simulink model "Compliance_Front_Axle_"  (R2026a)
settings: Solver=ode23t  StopTime=2
undefined symbols (not defined in the file or in its folder): Camber_Clearance_Coeff, Freeplay_Damping, Freeplay_Stiffness, Freeplay_Threshold, Jounce_Clearance_Coeff, Nominal_Clearance, Steer_Clearance_Coeff, X, Y, Z
libraries: sm_lib x5, nesl_utility x3
settings Model: Creator=Milán  LastModifiedBy=Milán

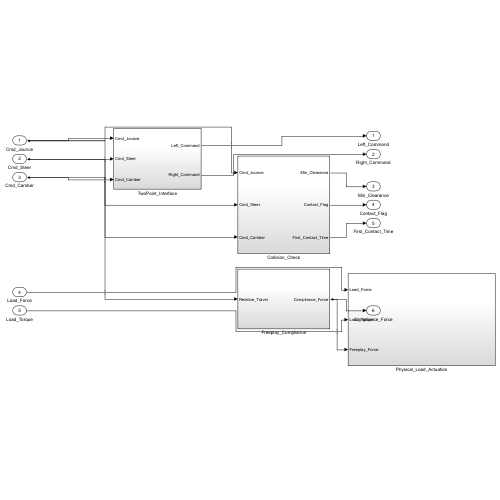
[thumbnail: Simulink's stored preview of the top-level diagram]
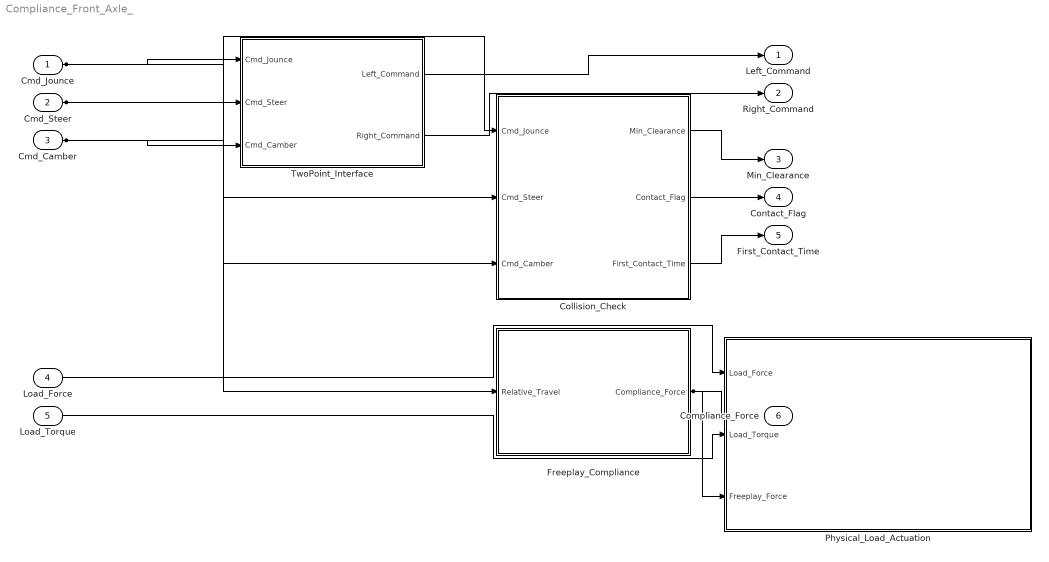
== system Compliance_Front_Axle_ ==
  Cmd_Jounce : Inport
  Cmd_Steer : Inport  Port=2
  Cmd_Camber : Inport  Port=3
  Load_Force : Inport  Port=4  PortDimensions=3
  Load_Torque : Inport  Port=5  PortDimensions=3
  Collision_Check : Subsystem
  Freeplay_Compliance : Subsystem
  Physical_Load_Actuation : Subsystem
  TwoPoint_Interface : Subsystem
  Left_Command : Outport
  Right_Command : Outport  Port=2
  Min_Clearance : Outport  Port=3
  Contact_Flag : Outport  Port=4
  First_Contact_Time : Outport  Port=5
  Compliance_Force : Outport  Port=6
  wires:
  Cmd_Jounce/1 -> TwoPoint_Interface/1(Cmd_Jounce), Collision_Check/1(Cmd_Jounce), Freeplay_Compliance/1(Relative_Travel)
  Cmd_Steer/1 -> TwoPoint_Interface/2(Cmd_Steer), Collision_Check/2(Cmd_Steer)
  Cmd_Camber/1 -> TwoPoint_Interface/3(Cmd_Camber), Collision_Check/3(Cmd_Camber)
  TwoPoint_Interface/1(Left_Command) -> Left_Command/1
  TwoPoint_Interface/2(Right_Command) -> Right_Command/1
  Collision_Check/1(Min_Clearance) -> Min_Clearance/1
  Collision_Check/2(Contact_Flag) -> Contact_Flag/1
  Collision_Check/3(First_Contact_Time) -> First_Contact_Time/1
  Freeplay_Compliance/1(Compliance_Force) -> Compliance_Force/1, Physical_Load_Actuation/3(Freeplay_Force)
  Load_Force/1 -> Physical_Load_Actuation/1(Load_Force)
  Load_Torque/1 -> Physical_Load_Actuation/2(Load_Torque)

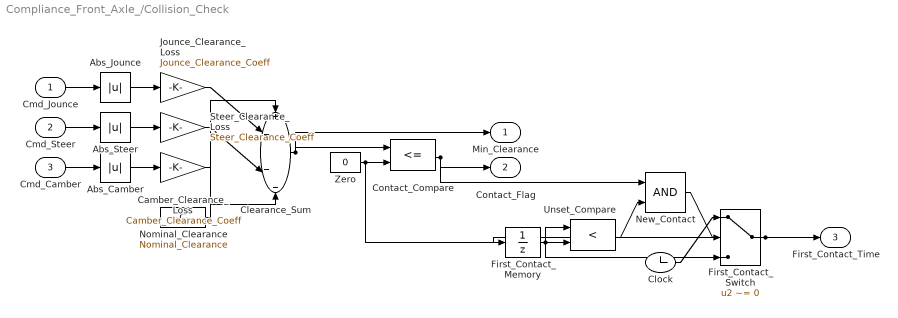
== system Compliance_Front_Axle_/Collision_Check ==
  Cmd_Jounce : Inport
  Cmd_Steer : Inport  Port=2
  Cmd_Camber : Inport  Port=3
  Abs_Camber : Abs  SaturateOnIntegerOverflow=off
  Abs_Jounce : Abs  SaturateOnIntegerOverflow=off
  Abs_Steer : Abs  SaturateOnIntegerOverflow=off
  Camber_Clearance_Loss : Gain  Gain=Camber_Clearance_Coeff
  Clearance_Sum : Sum  Inputs=+---
  Clock : Clock
  Contact_Compare : RelationalOperator  Operator=<=  OutDataTypeStr=boolean  RndMeth=Simplest  InputSameDT=off
  First_Contact_Memory : UnitDelay  InitialCondition=-1  SampleTime=-1
  First_Contact_Switch : Switch  Criteria=u2 ~= 0  SaturateOnIntegerOverflow=off  InputSameDT=off
  Jounce_Clearance_Loss : Gain  Gain=Jounce_Clearance_Coeff
  New_Contact : Logic  AllPortsSameDT=off  OutDataTypeStr=boolean
  Nominal_Clearance : Constant  Value=Nominal_Clearance
  Steer_Clearance_Loss : Gain  Gain=Steer_Clearance_Coeff
  Unset_Compare : RelationalOperator  Operator=<  OutDataTypeStr=boolean  RndMeth=Simplest  InputSameDT=off
  Zero : Constant  Value=0
  Min_Clearance : Outport
  Contact_Flag : Outport  Port=2
  First_Contact_Time : Outport  Port=3
  wires:
  Cmd_Jounce/1 -> Abs_Jounce/1
  Cmd_Steer/1 -> Abs_Steer/1
  Cmd_Camber/1 -> Abs_Camber/1
  Abs_Jounce/1 -> Jounce_Clearance_Loss/1
  Abs_Steer/1 -> Steer_Clearance_Loss/1
  Abs_Camber/1 -> Camber_Clearance_Loss/1
  Nominal_Clearance/1 -> Clearance_Sum/1
  Jounce_Clearance_Loss/1 -> Clearance_Sum/2
  Steer_Clearance_Loss/1 -> Clearance_Sum/3
  Camber_Clearance_Loss/1 -> Clearance_Sum/4
  Clearance_Sum/1 -> Min_Clearance/1, Contact_Compare/1
  Zero/1 -> Contact_Compare/2, Unset_Compare/2
  Contact_Compare/1 -> Contact_Flag/1, New_Contact/1
  First_Contact_Memory/1 -> Unset_Compare/1, First_Contact_Switch/3
  Unset_Compare/1 -> New_Contact/2
  Clock/1 -> First_Contact_Switch/1
  New_Contact/1 -> First_Contact_Switch/2
  First_Contact_Switch/1 -> First_Contact_Memory/1, First_Contact_Time/1

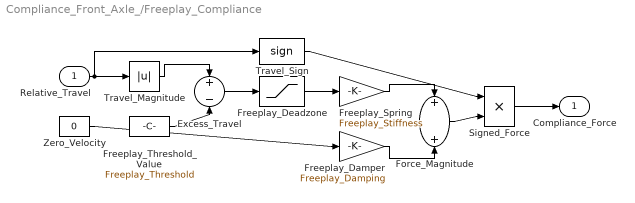
== system Compliance_Front_Axle_/Freeplay_Compliance ==
  Relative_Travel : Inport
  Excess_Travel : Sum  Inputs=+-
  Force_Magnitude : Sum
  Freeplay_Damper : Gain  Gain=Freeplay_Damping
  Freeplay_Deadzone : Saturate  UpperLimit=inf  LowerLimit=0
  Freeplay_Spring : Gain  Gain=Freeplay_Stiffness
  Freeplay_Threshold_Value : Constant  Value=Freeplay_Threshold
  Signed_Force : Product
  Travel_Magnitude : Abs  SaturateOnIntegerOverflow=off
  Travel_Sign : Signum
  Zero_Velocity : Constant  Value=0
  Compliance_Force : Outport
  wires:
  Relative_Travel/1 -> Travel_Magnitude/1, Travel_Sign/1
  Travel_Magnitude/1 -> Excess_Travel/1
  Freeplay_Threshold_Value/1 -> Excess_Travel/2
  Excess_Travel/1 -> Freeplay_Deadzone/1
  Freeplay_Deadzone/1 -> Freeplay_Spring/1
  Zero_Velocity/1 -> Freeplay_Damper/1
  Freeplay_Spring/1 -> Force_Magnitude/1
  Freeplay_Damper/1 -> Force_Magnitude/2
  Travel_Sign/1 -> Signed_Force/1
  Force_Magnitude/1 -> Signed_Force/2
  Signed_Force/1 -> Compliance_Force/1

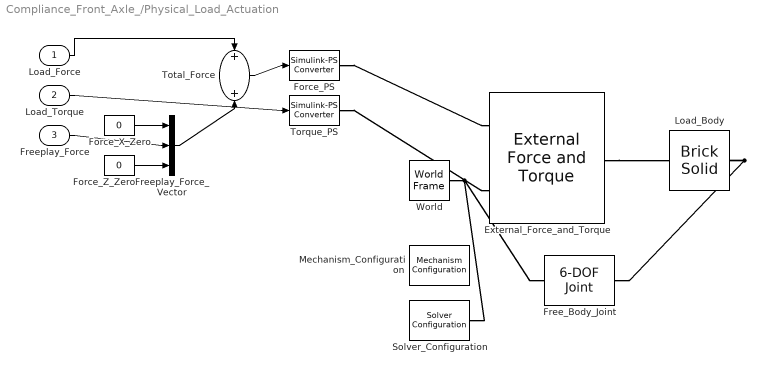
== system Compliance_Front_Axle_/Physical_Load_Actuation ==
  Load_Force : Inport  PortDimensions=3
  Load_Torque : Inport  Port=2  PortDimensions=3
  Freeplay_Force : Inport  Port=3
  External_Force_and_Torque : sm_lib/Forces and Torques/External Force and Torque  EnableForceX=off  EnableForceY=off  EnableForceZ=off  EnableForce=on  ForceResolutionFrame=AttachedFrame  EnableTorqueX=off  EnableTorqueY=off  EnableTorqueZ=off  EnableTorque=on  TorqueResolutionFrame=AttachedFrame
  Force_PS : nesl_utility/Simulink-PS Converter  PhysicalDomain=network_engine_domain  SubClassName=ps_input  LeftPortType=input  RightPortType=output  PseudoPeriodic=off  Frequencies=[]  NoiseDistribution=none  NoiseParameters=[]  Unit=1  AffineConversion=off  FilteringAndDerivatives=provide  SimscapeFilterOrder=1  InputFilterTimeConstant=0.001  UdotUserProvided=0
  Force_X_Zero : Constant  Value=0
  Force_Z_Zero : Constant  Value=0
  Free_Body_Joint : sm_lib/Joints/6-DOF Joint  JointMode=Normal  CompositeWrenchDir=FollowerOnBase  CompositeWrenchFrame=BaseFrame  SenseConstraintForce=off  SenseConstraintTorque=off  SenseTotalForce=off  SenseTotalTorque=off  PxPositionTargetSpecify=off  PxPositionTargetPriority=High  PxPositionTargetValue=0  PxPositionTargetValueUnits=m  PxVelocityTargetSpecify=off  PxVelocityTargetPriority=High  PxVelocityTargetValue=0  PxVelocityTargetValueUnits=m/s  PxEquilibriumPosition=0  PxEquilibriumPositionUnits=m  PxSpringStiffness=0  PxSpringStiffnessUnits=N/m  PxDampingCoefficient=0  PxDampingCoefficientUnits=N/(m/s)  PxLowerLimitSpecify=off  PxLowerLimitBound=-1  PxLowerLimitBoundUnits=m  PxLowerLimitStiffness=1e6  PxLowerLimitStiffnessUnits=N/m  PxLowerLimitDamping=1e3  PxLowerLimitDampingUnits=N/(m/s)  PxLowerLimitTransitionRegionWidth=1e-4  PxLowerLimitTransitionRegionWidthUnits=m  PxUpperLimitSpecify=off  PxUpperLimitBound=1  PxUpperLimitBoundUnits=m  PxUpperLimitStiffness=1e6  PxUpperLimitStiffnessUnits=N/m  PxUpperLimitDamping=1e3  PxUpperLimitDampingUnits=N/(m/s)  PxUpperLimitTransitionRegionWidth=1e-4  PxUpperLimitTransitionRegionWidthUnits=m  PxTorqueActuationMode=NoTorque  PxMotionActuationMode=ComputedMotion  PxSensePosition=off  PxSenseVelocity=off  PxSenseAcceleration=off  PxSenseTorqueForce=off  PxSenseLowerLimitTorqueForce=off  PxSenseUpperLimitTorqueForce=off  PyPositionTargetSpecify=off  PyPositionTargetPriority=High  PyPositionTargetValue=0  PyPositionTargetValueUnits=m  PyVelocityTargetSpecify=off  PyVelocityTargetPriority=High  PyVelocityTargetValue=0  PyVelocityTargetValueUnits=m/s  PyEquilibriumPosition=0  PyEquilibriumPositionUnits=m  PySpringStiffness=0  PySpringStiffnessUnits=N/m  PyDampingCoefficient=0  PyDampingCoefficientUnits=N/(m/s)  PyLowerLimitSpecify=off  PyLowerLimitBound=-1  PyLowerLimitBoundUnits=m  PyLowerLimitStiffness=1e6  PyLowerLimitStiffnessUnits=N/m  PyLowerLimitDamping=1e3  PyLowerLimitDampingUnits=N/(m/s)  PyLowerLimitTransitionRegionWidth=1e-4  PyLowerLimitTransitionRegionWidthUnits=m  PyUpperLimitSpecify=off  PyUpperLimitBound=1  PyUpperLimitBoundUnits=m  PyUpperLimitStiffness=1e6  PyUpperLimitStiffnessUnits=N/m  PyUpperLimitDamping=1e3  PyUpperLimitDampingUnits=N/(m/s)  PyUpperLimitTransitionRegionWidth=1e-4  PyUpperLimitTransitionRegionWidthUnits=m  PyTorqueActuationMode=NoTorque  PyMotionActuationMode=ComputedMotion  PySensePosition=off  PySenseVelocity=off  PySenseAcceleration=off  PySenseTorqueForce=off  PySenseLowerLimitTorqueForce=off  PySenseUpperLimitTorqueForce=off  PzPositionTargetSpecify=off  PzPositionTargetPriority=High  PzPositionTargetValue=0  PzPositionTargetValueUnits=m  PzVelocityTargetSpecify=off  PzVelocityTargetPriority=High  PzVelocityTargetValue=0  PzVelocityTargetValueUnits=m/s  PzEquilibriumPosition=0  PzEquilibriumPositionUnits=m  PzSpringStiffness=0  PzSpringStiffnessUnits=N/m  PzDampingCoefficient=0  PzDampingCoefficientUnits=N/(m/s)  PzLowerLimitSpecify=off  PzLowerLimitBound=-1  PzLowerLimitBoundUnits=m  PzLowerLimitStiffness=1e6  PzLowerLimitStiffnessUnits=N/m  PzLowerLimitDamping=1e3  PzLowerLimitDampingUnits=N/(m/s)  PzLowerLimitTransitionRegionWidth=1e-4  PzLowerLimitTransitionRegionWidthUnits=m  PzUpperLimitSpecify=off  PzUpperLimitBound=1  PzUpperLimitBoundUnits=m  PzUpperLimitStiffness=1e6  PzUpperLimitStiffnessUnits=N/m  PzUpperLimitDamping=1e3  PzUpperLimitDampingUnits=N/(m/s)  PzUpperLimitTransitionRegionWidth=1e-4  PzUpperLimitTransitionRegionWidthUnits=m  PzTorqueActuationMode=NoTorque  PzMotionActuationMode=ComputedMotion  PzSensePosition=off  PzSenseVelocity=off  PzSenseAcceleration=off  PzSenseTorqueForce=off  PzSenseLowerLimitTorqueForce=off  PzSenseUpperLimitTorqueForce=off  SphPositionTargetSpecify=off  SphPositionTargetPriority=High  SphPositionTargetRotationMethod=None  SphPositionTargetFollAlignAxisA=+X  SphPositionTargetBaseAlignAxisA=+Y  SphPositionTargetFollAlignAxisB=+Y  SphPositionTargetBaseAlignAxisB=+Z  SphPositionTargetRotationStandardAxis=+Z  SphPositionTargetRotationAngle=0  SphPositionTargetRotationAngleUnits=deg  SphPositionTargetRotationArbitraryAxis=[0 0 1]  SphPositionTargetRotationSequenceAxes=FollowerAxes  SphPositionTargetRotationSequence=XYX  SphPositionTargetRotationSequenceAngles=[0 0 0]  SphPositionTargetRotationSequenceAnglesUnits=deg  SphPositionTargetRotationMatrix=[1 0 0;0 1 0;0 0 1]  SphPositionTargetQuaternion=[1 0 0 0]  SphVelocityTargetSpecify=off  SphVelocityTargetPriority=High  SphVelocityTargetValue=[0 0 0]  SphVelocityTargetValueUnits=deg/s  SphVelocityTargetInFollowerFrame=on  SphEqPosRotationMethod=None  SphEqPosFollAlignAxisA=+X  SphEqPosBaseAlignAxisA=+Y  SphEqPosFollAlignAxisB=+Y  SphEqPosBaseAlignAxisB=+Z  SphEqPosRotationStandardAxis=+Z  SphEqPosRotationAngle=0  SphEqPosRotationAngleUnits=deg  SphEqPosRotationArbitraryAxis=[0 0 1]  SphEqPosRotationSequenceAxes=FollowerAxes  SphEqPosRotationSequence=XYX  SphEqPosRotationSequenceAngles=[0 0 0]  SphEqPosRotationSequenceAnglesUnits=deg  SphEqPosRotationMatrix=[1 0 0;0 1 0;0 0 1]  SphEqPosQuaternion=[1 0 0 0]  SphSpringStiffness=0  SphSpringStiffnessUnits=N*m/deg  SphDampingCoefficient=0  SphDampingCoefficientUnits=N*m/(deg/s)  SphLowerLimitSpecify=off  SphLowerLimitBound=15  SphLowerLimitBoundUnits=deg  SphLowerLimitStiffness=1e4  SphLowerLimitStiffnessUnits=N*m/deg  SphLowerLimitDamping=10  SphLowerLimitDampingUnits=N*m/(deg/s)  SphLowerLimitTransitionRegionWidth=0.1  SphLowerLimitTransitionRegionWidthUnits=deg  SphUpperLimitSpecify=off  SphUpperLimitBound=45  SphUpperLimitBoundUnits=deg  SphUpperLimitStiffness=1e4  SphUpperLimitStiffnessUnits=N*m/deg  SphUpperLimitDamping=10  SphUpperLimitDampingUnits=N*m/(deg/s)  SphUpperLimitTransitionRegionWidth=0.1  SphUpperLimitTransitionRegionWidthUnits=deg  SphTorqueActuationMode=NoTorque  SphActuateTorqueX=off  SphActuateTorqueY=off  SphActuateTorqueZ=off  SphActuateTorque=off  SphActuationFrame=BaseFrame  SphSensePosition=off  SphSenseVelocityX=off  SphSenseVelocityY=off  SphSenseVelocityZ=off  SphSenseVelocity=off  SphSenseAccelerationX=off  SphSenseAccelerationY=off  SphSenseAccelerationZ=off  SphSenseAcceleration=off  SphSenseLowerLimitTorqueMag=off  SphSenseUpperLimitTorqueMag=off  SphSensingFrame=BaseFrame
  Freeplay_Force_Vector : Mux  Inputs=3
  Load_Body : sm_lib/Body Elements/Brick Solid  BrickDimensions=[1 1 1]  BrickDimensionsUnits=m  ExportEntireGeometry=off  InertiaType=CalculateFromGeometry  BasedOnType=Density  Density=1000  DensityUnits=kg/m^3  Mass=1  MassUnits=kg  CenterOfMass=[0 0 0]  CenterOfMassUnits=m  MomentsOfInertia=[1 1 1]  MomentsOfInertiaUnits=kg*m^2  ProductsOfInertia=[0 0 0]  ProductsOfInertiaUnits=kg*m^2  GraphicType=FromGeometry  MarkerShape=Sphere  MarkerSize=10  GraphicVisPropType=SimpleVisualProperties  GraphicDiffuseColor=[0.5 0.5 0.5]  GraphicOpacity=1  GraphicSpecularColor=[0.5 0.5 0.5 1.0]  GraphicAmbientColor=[0.15 0.15 0.15 1.0]  GraphicEmissiveColor=[0.0 0.0 0.0 1.0]  GraphicShininess=75  DoExposeReferenceFrame=on  SerializedFrames=<Frames/>
  Mechanism_Configuration : sm_lib/Utilities/Mechanism Configuration  UniformGravity=Constant  GravityVector=[0 0 -9.80665]  GravityVectorUnits=m/s^2  LinearizationDelta=0.001  JointModeTransitionNonlinearIterations=2
  Solver_Configuration : nesl_utility/Solver Configuration  PhysicalDomain=network_engine_domain  SubClassName=solver  LeftPortType=input  RightPortType=generic  Tones=[]  Harmonics=[]  SimulateNoise=off  Profile=off  UseLocalSampling=off  EnableSwitchedLinearOptims=on  FrequencyDomain=off  UseCCode=off  RelTol=0.001  AbsTol=0.001  MinStep=1e-09  ToWorkspace=off  RevertToSquareIcSolve=off  NumHomotopyIterations=100  PhasorMode=off  PhasorModeNumHarmonics=1  ConsistencySolver=NEWTON_XTOL_AFTER_FTOL  CanonicalOrdering=CANONICAL  OptimizeIntermediates=OPTIMIZED  IndexReductionMethod=DerivativeReplacement  DoDC=off  ResidualTolerance=1e-09  ConsistencyTolSource=GLOBAL  ConsistencyAbsTol=0.001  ConsistencyRelTol=0.001  ConsistencyTolFactor=0.001  UseLocalSolver=off  LocalSolverChoice=NE_BACKWARD_EULER_ADVANCER  ResolveIndetEquations=on  FunctionEvalNumThread=1  LocalSolverSampleTime=0.001  DoFixedCost=off  MaxNonlinIter=3  MaxModeIter=2  ComputeImpulses=off  ImpulseIterations=2  LinearAlgebra=auto  LinearAlgebraNumThread=0  EquationFormulation=NE_TIME_EF  DelaysMemoryBudget=1024  AutomaticFiltering=on  FilteringTimeConstant=0.001  PartitionStorageMethod=AS_NEEDED  PartitionMemoryBudget=1024  PartitionMethod=ROBUST  MultibodyUseLocalSolver=off  MultibodyLocalSolverChoice=ODE1  MultibodyLocalSolverSampleTime=0.001
  Torque_PS : nesl_utility/Simulink-PS Converter  PhysicalDomain=network_engine_domain  SubClassName=ps_input  LeftPortType=input  RightPortType=output  PseudoPeriodic=off  Frequencies=[]  NoiseDistribution=none  NoiseParameters=[]  Unit=1  AffineConversion=off  FilteringAndDerivatives=provide  SimscapeFilterOrder=1  InputFilterTimeConstant=0.001  UdotUserProvided=0
  Total_Force : Sum
  World : sm_lib/Frames and Transforms/World Frame
  wires:
  Force_X_Zero/1 -> Freeplay_Force_Vector/1
  Freeplay_Force/1 -> Freeplay_Force_Vector/2
  Force_Z_Zero/1 -> Freeplay_Force_Vector/3
  Load_Force/1 -> Total_Force/1
  Freeplay_Force_Vector/1 -> Total_Force/2
  Total_Force/1 -> Force_PS/1
  Load_Torque/1 -> Torque_PS/1
  connections:
  Force_PS/RConn1 -- External_Force_and_Torque/LConn1
  Torque_PS/RConn1 -- External_Force_and_Torque/LConn2
  Free_Body_Joint/LConn1 -- World/RConn1 -- Solver_Configuration/RConn1
  Load_Body/RConn1 -- Free_Body_Joint/RConn1 -- External_Force_and_Torque/RConn1

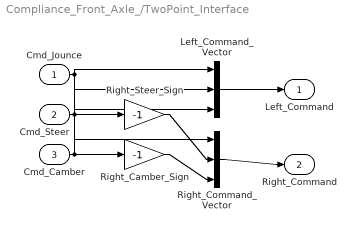
== system Compliance_Front_Axle_/TwoPoint_Interface ==
  Cmd_Jounce : Inport
  Cmd_Steer : Inport  Port=2
  Cmd_Camber : Inport  Port=3
  Left_Command_Vector : Mux  Inputs=3
  Right_Camber_Sign : Gain  Gain=-1
  Right_Command_Vector : Mux  Inputs=3
  Right_Steer_Sign : Gain  Gain=-1
  Left_Command : Outport
  Right_Command : Outport  Port=2
  wires:
  Cmd_Jounce/1 -> Left_Command_Vector/1, Right_Command_Vector/1
  Cmd_Steer/1 -> Left_Command_Vector/2, Right_Steer_Sign/1
  Cmd_Camber/1 -> Left_Command_Vector/3, Right_Camber_Sign/1
  Right_Steer_Sign/1 -> Right_Command_Vector/2
  Right_Camber_Sign/1 -> Right_Command_Vector/3
  Left_Command_Vector/1 -> Left_Command/1
  Right_Command_Vector/1 -> Right_Command/1
